simulink model "New_BMS_2"  (R2023b)
settings: Solver=FixedStepAuto  StartTime=0.0  StopTime=1000  FixedStep=0.1  RelTol=1e-3
InitFcn:
  | mbd_s32k_consistency_checks(bdroot(gcs));
undefined symbols (not defined in the file or in its folder): DiscIntNeverNeededParam, LQFP
libraries: mbd_s32k1xx_ec_toolbox x12, simulink x1
settings Model: Creator=snith  LastModifiedBy=HP
settings DataIOCC: ExternalInput=off  InitialState=off  SaveOutput=off  SignalLogging=off  SaveTime=off
settings OptimizationCC: DefaultParameterBehavior=Inlined  EnhancedBackFolding=on  PassReuseOutputArgsAs=Individual arguments  ZeroExternalMemoryAtStartup=off  ZeroInternalMemoryAtStartup=off  OptimizeBlockOrder=speed  DifferentSizesBufferReuse=on  OptimizationCustomize=off  EfficientTunableParamExpr=on
settings DebuggingCC: InheritedTsInSrcMsg=none  SingleTaskRateTransMsg=error  ParameterTunabilityLossMsg=error  UnconnectedInputMsg=error  UnconnectedOutputMsg=error  UnconnectedLineMsg=error  UnknownTsInhSupMsg=error
settings HardwareCC: ProdBitPerPointer=32  ProdBitPerSizeT=32  ProdBitPerPtrDiffT=32  ProdLargestAtomicInteger=Long  ProdLargestAtomicFloat=Double  ProdWordSize=32  ProdHWDeviceType=ARM Compatible->ARM Cortex
settings SFSimCC: MATLABDynamicMemAlloc=off
settings RTWCC: Description=Model Based Design Toolbox S32K1xx Code Generation Target  SystemTargetFile=mbd_s32k.tlc  MakeCommand=mbd_s32k_make_rtw COPY_MDLREF_INCLUDES=0  TemplateMakefile=mbd_s32k.tmf
settings CodeAppCC: ForceParamTrailComments=on  IgnoreCustomStorageClasses=off  OperatorAnnotations=on  SimulinkDataObjDesc=on  SFDataObjDesc=on  InsertBlockDesc=on
settings STFCustomTargetCC: MultiwordLength=256  CombineOutputUpdateFcns=on  ERTCustomFileBanners=on  SupportContinuousTime=off  SupportNonInlinedSFcns=off  RemoveResetFunc=on  MATLABClassNameForMDSCustomization=Simulink.SoftwareTarget.ERTCustomization  SystemTargetFile=mbd_s32k.tlc
settings ERTTargetCC: TargetLangStandard=C99 (ISO)  ParMdlRefBuildCompliant=off  CompOptLevelCompliant=off  ConcurrentExecutionCompliant=off  ModelStepFunctionPrototypeControlCompliant=off  CPPClassGenCompliant=off  UseToolchainInfoCompliant=off  InlinedParameterPlacement=NonHierarchical  ERTSrcFileBannerTemplate=mbd_ert_code_template.cgt  ERTHdrFileBannerTemplate=mbd_ert_code_template.cgt  ERTDataSrcFileTemplate=mbd_ert_code_template.cgt  ERTDataHdrFileTemplate=mbd_ert_code_template.cgt  ERTCustomFileTemplate=example_file_process.tlc
settings ConfigComp: CovBoundaryAbsTol=1.0e-5

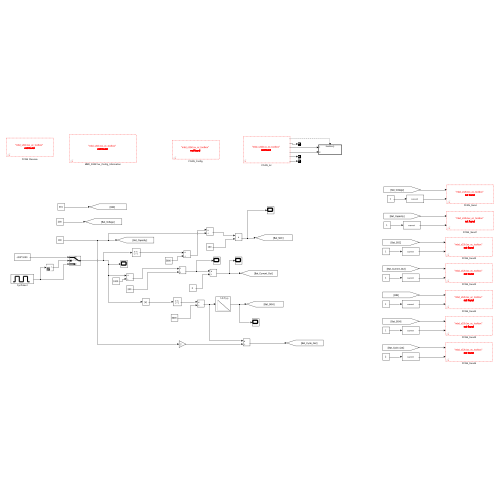
[thumbnail: Simulink's stored preview of the top-level diagram]
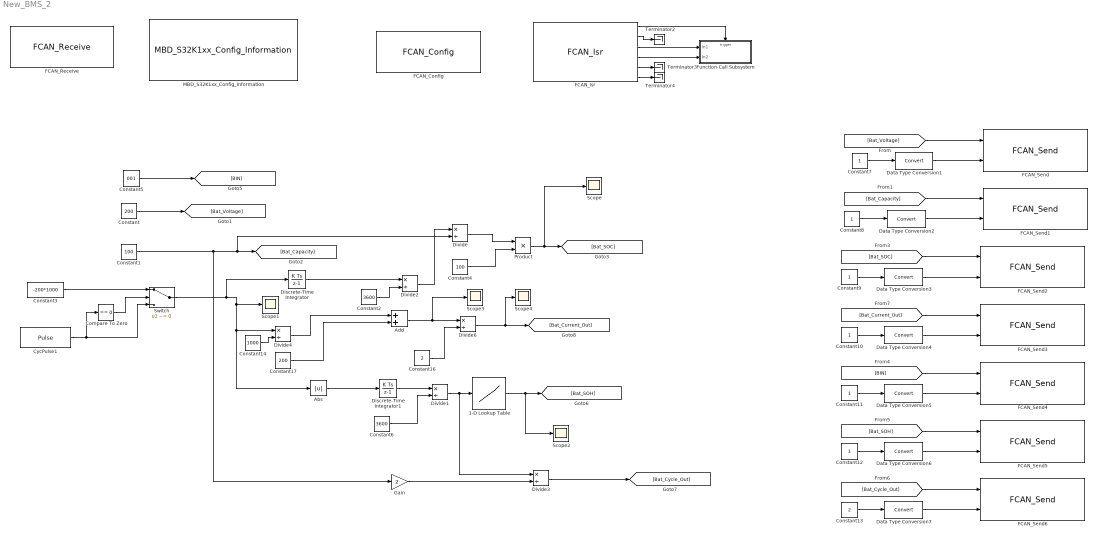
== system New_BMS_2 ==
  1-D Lookup Table : Lookup_n-D  NumberOfTableDimensions=1  BreakpointsForDimension1=[0 10000 20000 40000 60000 80000 100000 120000 140000 160000 180000]  Table=[100 99 98 96 94 92 90 88 86 84 82]  TableDataTypeStr=Inherit: Inherit from 'Table data'  ExtrapMethod=Clip  InternalRulePriority=Speed  OutDataTypeStr=uint8  RndMeth=Simplest
  Abs : Abs  SaturateOnIntegerOverflow=off
  Add : Sum  OutDataTypeStr=Inherit: Inherit via back propagation
  Compare To Zero : simulink/Logic and Bit Operations/Compare To Zero  relop===  OutDataTypeStr=boolean
  Constant : Constant  Value=200  OutDataTypeStr=uint8
  Constant1 : Constant  Value=100  OutDataTypeStr=uint8
  Constant{7..12} (6 alike) : Constant
  Constant13 : Constant  Value=2
  Constant14 : Constant  Value=1000
  Constant16 : Constant  Value=2
  Constant17 : Constant  Value=200
  Constant2 : Constant  Value=3600
  Constant3 : Constant  Value=-200*1000
  Constant4 : Constant  Value=100
  Constant5 : Constant  Value=001  OutDataTypeStr=uint8
  Constant6 : Constant  Value=3600
  CycPulse1 : DiscretePulseGenerator  PulseType=Time based  Amplitude=200*1000  Period=3600/1000  PulseWidth=50
  Data Type Conversion{1..7} (7 alike) : DataTypeConversion  SaturateOnIntegerOverflow=off  RndMeth=Floor
  Discrete-Time Integrator : DiscreteIntegrator  SampleTime=-1  ICPrevOutput=DiscIntNeverNeededParam  ICPrevScaledInput=DiscIntNeverNeededParam
  Discrete-Time Integrator1 : DiscreteIntegrator  SampleTime=-1  ICPrevOutput=DiscIntNeverNeededParam  ICPrevScaledInput=DiscIntNeverNeededParam
  Divide : Product  Inputs=*/
  Divide1 : Product  Inputs=*/
  Divide2 : Product  Inputs=*/
  Divide3 : Product  Inputs=*/  OutDataTypeStr=uint8
  Divide4 : Product  Inputs=*/  OutDataTypeStr=double
  Divide6 : Product  Inputs=*/  OutDataTypeStr=uint8
  FCAN_Config : mbd_s32k1xx_ec_toolbox/Communication Blocks/CAN Blocks/FCAN_Config  Priority=1  can_instance=0  can_mode=Normal mode  can_max_num_mb=20  can_rx=PTE4: [CAN0_RX | CAN Rx channel]  can_tx=PTE5: [CAN0_TX | CAN Tx Channel]  show_adv_opts=on  can_clk_src=Peripheral clock  can_clk_freq=80 MHz  bitrate_to_time_seg=on  bitrate=500  sample_point=80  real_bitrate=500  real_sample_point=80  prop_delay=250  bus_length=1  tq=200.0  time_quanta=10  can_presdiv=16  can_propseg=3  can_pseg1=4  can_pseg2=2  can_rjw=2  cbt_bitrate=2000  cbt_sample_point=80  cbt_real_bitrate=2000  cbt_real_sample_point=80  cbt_tq=25.0  cbt_time_quanta=40  can_cbt_presdiv=2  can_cbt_propseg=29  can_cbt_pseg1=5  can_cbt_pseg2=5  can_cbt_rjw=5  can_fd_enable=off  can_payload=8  tdc_enable=off  tdc_offset=20  can_rxfifo_enable=off  can_num_id_filters=8  can_fifo_id_format=A  can_fifo_id_filter={{false,false,'0x0'},{false,false,'0x0'},{false,false,'0x0'},{false,false,'0x0'},{false,false,'0x0'},{false,false,'0x0'},{false,false,'0x0'},{false,false,'0x0'}}  can_pn_enable=off  can_wakeup_match=off  can_wakeup_timeout=off  can_timeout_en=off  can_match_timeout=1  can_multiple_matches_en=off  can_num_matches=1  can_idfilter_extendedid=off  can_idfilter_remoteframe=off  can_idfilter_type=Match exact  can_idfilter_id1=0  can_idfilter_id2=0  can_payloadfilter_enable=off  can_payloadfilter_dlclow=0  can_payloadfilter_dlchigh=0  can_payloadfilter_type=Match exact  can_payloadfilter_payload1_b0=0  can_payloadfilter_payload1_b1=0  can_payloadfilter_payload1_b2=0  can_payloadfilter_payload1_b3=0  can_payloadfilter_payload1_b4=0  can_payloadfilter_payload1_b5=0  can_payloadfilter_payload1_b6=0  can_payloadfilter_payload1_b7=0  can_payloadfilter_payload2_b0=0  can_payloadfilter_payload2_b1=0  can_payloadfilter_payload2_b2=0  can_payloadfilter_payload2_b3=0  can_payloadfilter_payload2_b4=0  can_payloadfilter_payload2_b5=0  can_payloadfilter_payload2_b6=0  can_payloadfilter_payload2_b7=0
  FCAN_Isr : mbd_s32k1xx_ec_toolbox/Communication Blocks/CAN Blocks/FCAN_Isr  can_instance=0  can_event=Rx Complete
  FCAN_Receive : mbd_s32k1xx_ec_toolbox/Communication Blocks/CAN Blocks/FCAN_Receive  can_instance=0  can_mode=Non-blocking  can_timeout_ms=0  can_mb_idx=19  can_mb_init=Once  show_id_input=off  can_extended_id=off  can_is_remote=off  can_id=123  can_msg_mask=FFFFFFFF  show_adv_opts=off  can_use_rxfifo=off  can_fd_enable=off
  FCAN_Send : mbd_s32k1xx_ec_toolbox/Communication Blocks/CAN Blocks/FCAN_Send  can_instance=0  can_mode=Non-blocking  can_timeout_ms=0  can_mb_idx=10  can_mb_init=On each call  show_id_input=off  can_extended_id=off  can_is_remote=off  can_id=100  show_adv_opts=off  can_fd_enable=off  can_enable_brs=off  can_fd_padding=0
  FCAN_Send1 : mbd_s32k1xx_ec_toolbox/Communication Blocks/CAN Blocks/FCAN_Send  can_instance=0  can_mode=Non-blocking  can_timeout_ms=0  can_mb_idx=11  can_mb_init=On each call  show_id_input=off  can_extended_id=off  can_is_remote=off  can_id=101  show_adv_opts=off  can_fd_enable=off  can_enable_brs=off  can_fd_padding=0
  FCAN_Send2 : mbd_s32k1xx_ec_toolbox/Communication Blocks/CAN Blocks/FCAN_Send  can_instance=0  can_mode=Non-blocking  can_timeout_ms=0  can_mb_idx=12  can_mb_init=On each call  show_id_input=off  can_extended_id=off  can_is_remote=off  can_id=102  show_adv_opts=off  can_fd_enable=off  can_enable_brs=off  can_fd_padding=0
  FCAN_Send3 : mbd_s32k1xx_ec_toolbox/Communication Blocks/CAN Blocks/FCAN_Send  can_instance=0  can_mode=Non-blocking  can_timeout_ms=0  can_mb_idx=13  can_mb_init=On each call  show_id_input=off  can_extended_id=off  can_is_remote=off  can_id=103  show_adv_opts=off  can_fd_enable=off  can_enable_brs=off  can_fd_padding=0
  FCAN_Send4 : mbd_s32k1xx_ec_toolbox/Communication Blocks/CAN Blocks/FCAN_Send  can_instance=0  can_mode=Non-blocking  can_timeout_ms=0  can_mb_idx=14  can_mb_init=On each call  show_id_input=off  can_extended_id=off  can_is_remote=off  can_id=104  show_adv_opts=off  can_fd_enable=off  can_enable_brs=off  can_fd_padding=0
  FCAN_Send5 : mbd_s32k1xx_ec_toolbox/Communication Blocks/CAN Blocks/FCAN_Send  can_instance=0  can_mode=Non-blocking  can_timeout_ms=0  can_mb_idx=15  can_mb_init=On each call  show_id_input=off  can_extended_id=off  can_is_remote=off  can_id=105  show_adv_opts=off  can_fd_enable=off  can_enable_brs=off  can_fd_padding=0
  FCAN_Send6 : mbd_s32k1xx_ec_toolbox/Communication Blocks/CAN Blocks/FCAN_Send  can_instance=0  can_mode=Non-blocking  can_timeout_ms=0  can_mb_idx=16  can_mb_init=On each call  show_id_input=off  can_extended_id=off  can_is_remote=off  can_id=106  show_adv_opts=off  can_fd_enable=off  can_enable_brs=off  can_fd_padding=0
  Function-Call Subsystem : Subsystem  TreatAsAtomicUnit=on
  Gain : Gain  Gain=2
  MBD_S32K1xx_Config_Information : mbd_s32k1xx_ec_toolbox/MBD_S32K1xx_Config_Information  mbdt_ver=0  disp_str=|  config_params=[]  mcu_target_name=S32K144  mcu_target_package=100-LQFP  mcu_target_sram_size=48KB  mcu_system_clock_freq=80  mcu_xtal_freq=External 8  mcu_steptick_timer=LPIT Channel 0  mcu_steptick_prio=15  ds_import_enable=on  target_compiler=GCC  target_memory=FLASH  gcc_target_compile_opts=-mthumb -mfloat-abi=hard -mfpu=fpv4-sp-d16 -O1 -g -gstrict-dwarf  gcc_target_assemble_opts=-mthumb -mfloat-abi=hard -mfpu=fpv4-sp-d16 -g  gcc_target_link_opts=-mthumb -mfloat-abi=hard -mfpu=fpv4-sp-d16  gcc_target_default_lcf=on  gcc_target_user_lcf=S32K144_48_flash.ld  ghs_target_compile_opts=-cpu=cortexm4f -thumb -fpu=vfpv4_d16 -fsingle -Ogeneral -Wundef -Wimplicit-int -Wshadow -Wtrigraphs --no_commons --gnu_asm -gnu99 -gdwarf-2 -G  ghs_target_assemble_opts=-cpu=cortexm4f -fpu=vfpv4_d16  ghs_target_link_opts=-cpu=cortexm4f -thumb -fpu=vfpv4_d16  ghs_target_default_lcf=on  ghs_target_user_lcf=S32K144_48_flash.ld  iar_target_compile_opts=--cpu=Cortex-M4F --thumb --fpu=VFPv4_sp -Ol -e --debug --dlib_config normal  iar_target_assemble_opts=--cpu Cortex-M4F --thumb --fpu VFPv4_sp  iar_target_link_opts=--no_exceptions --vfe --inline  iar_target_default_lcf=on  iar_target_user_lcf=S32K144_48_flash.icf  pil_download_enable=on  rbl_download_enable=on  rbl_start_delay=5000  rbl_download_interface=JTAG  rbl_restart_request=off  rbl_com_port=Custom  rbl_com_port_custom=COM1  pil_download_rate=57600  pil_download_rate_custom=115200  pil_opensda_drive=Custom  pil_opensda_drive_custom=D  jtag_interface=SEGGER JLink  jlink_default_path=off  jlink_user_path=C:\NXP\S32DS.3.5\Drivers\Segger  pil_uart_instance=1  pil_uart_rx=PTC6: [LPUART1_RX | Receive]  pil_uart_tx=PTC7: [LPUART1_TX | Transmit]  FTM_PWM_PcrCheckEnDis=on  FTM_Input_Edge_Inputs_PcrCheckEnDis=on  FTM_Dual_Edge_Inputs_PcrCheckEnDis=on  FTM_Quadrature_Inputs_PcrCheckEnDis=on  FTM_Hall_Sensor_Inputs_PcrCheckEnDis=on  LPTMR_PcrCheckEnDis=on  PIT_PcrCheckEnDis=on  RTC_PcrCheckEnDis=on  FlexCAN_PcrCheckEnDis=on  LIN_PcrCheckEnDis=on  FlexIO_PcrCheckEnDis=on  LPI2C_PcrCheckEnDis=on  LPSPI_PcrCheckEnDis=on  LPUART_PcrCheckEnDis=on  CMP_PcrCheckEnDis=on  GPIO_OutputPcrCheckEnDis=on  GPIO_InputPcrCheckEnDis=on  SBC_PcrCheckEnDis=on  BMS_PcrCheckEnDis=on  AMMCLIB_PcrCheckEnDis=on  FM_PcrCheckEnDis=on  Profile_PcrCheckEnDis=on  ConfigParams_PcrCheckEnDis=on  ModelRef_PcrCheckEnDis=on  PDB0_PcrCheckEnDis=on  CSEc_PcrCheckEnDis=on  eDMA_PcrCheckEnDis=on  FLASH_PcrCheckEnDis=on  ADC_PcrCheckEnDis=on  WDOG_PcrCheckEnDis=on
      | Target : S32K144-64KB_SRAM
      | Package : 100-pin
      | System clock : 80 MHz
      | XTAL clock : External 8 MHz
      | Compiler : IAR
      | Target Type : FLASH
      | Download Code after build : off
      | Step Tick Interrupt Priority : 15
  Product : Product  OutDataTypeStr=uint8
  Scope{,1..4} (5 alike) : Scope
  Switch : Switch  Criteria=u2 ~= 0  OutDataTypeStr=Inherit: Inherit via back propagation  SaturateOnIntegerOverflow=off  InputSameDT=off
  Terminator2 : Terminator
  Terminator3 : Terminator
  Terminator4 : Terminator
  wires:
  Switch/1 -> Discrete-Time Integrator/1, Scope1/1, Divide4/1, Abs/1
  Divide/1 -> Product/1
  Discrete-Time Integrator1/1 -> Divide1/1
  CycPulse1/1 -> Compare To Zero/1, Switch/3
  1-D Lookup Table/1 -> [Bat_SOH], Scope2/1
  Constant1/1 -> [Bat_Capacity], Divide/2, Gain/1
  Constant5/1 -> [BIN]
  Constant4/1 -> Product/2
  Discrete-Time Integrator/1 -> Divide2/1
  Constant6/1 -> Divide1/2
  Constant2/1 -> Divide2/2
  Constant3/1 -> Switch/1
  Compare To Zero/1 -> Switch/2
  Abs/1 -> Discrete-Time Integrator1/1
  Product/1 -> Scope/1, [Bat_SOC]
  Divide1/1 -> Divide3/1, 1-D Lookup Table/1
  Divide2/1 -> Divide/1
  Constant7/1 -> Data Type Conversion1/1
  Data Type Conversion1/1 -> FCAN_Send/2
  Gain/1 -> Divide3/2
  FCAN_Isr/3 -> Function-Call Subsystem/1(In1)
  FCAN_Isr/1 -> Function-Call Subsystem/Trigger
  FCAN_Isr/4 -> Function-Call Subsystem/2(In2)
  FCAN_Isr/2 -> Terminator2/1
  FCAN_Isr/5 -> Terminator3/1
  FCAN_Isr/6 -> Terminator4/1
  Constant/1 -> [Bat_Voltage]
  [Bat_Voltage] -> FCAN_Send/1
  [Bat_Capacity] -> FCAN_Send1/1
  Data Type Conversion2/1 -> FCAN_Send1/2
  Constant8/1 -> Data Type Conversion2/1
  Data Type Conversion3/1 -> FCAN_Send2/2
  [Bat_SOC] -> FCAN_Send2/1
  Constant9/1 -> Data Type Conversion3/1
  [Bat_Current_Out] -> FCAN_Send3/1
  Data Type Conversion4/1 -> FCAN_Send3/2
  Constant10/1 -> Data Type Conversion4/1
  Constant11/1 -> Data Type Conversion5/1
  [BIN] -> FCAN_Send4/1
  Data Type Conversion5/1 -> FCAN_Send4/2
  [Bat_SOH] -> FCAN_Send5/1
  Constant12/1 -> Data Type Conversion6/1
  Data Type Conversion6/1 -> FCAN_Send5/2
  Constant13/1 -> Data Type Conversion7/1
  Data Type Conversion7/1 -> FCAN_Send6/2
  [Bat_Cycle_Out] -> FCAN_Send6/1
  Constant14/1 -> Divide4/2
  Divide4/1 -> Add/1
  Divide3/1 -> [Bat_Cycle_Out]
  Constant17/1 -> Add/2
  Constant16/1 -> Divide6/2
  Add/1 -> Scope3/1, Divide6/1
  Divide6/1 -> Scope4/1, [Bat_Current_Out]

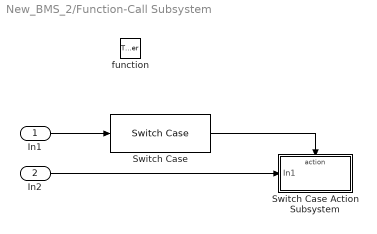
== system New_BMS_2/Function-Call Subsystem ==
  In1 : Inport
  In2 : Inport  Port=2
  function : TriggerPort  TriggerType=function-call  VariantControl=(inherit)
  Switch Case : SwitchCase  CaseConditions={hex2dec('123')}  ShowDefaultCase=off
  Switch Case Action Subsystem : Subsystem  TreatAsAtomicUnit=on
  wires:
  In1/1 -> Switch Case/1
  Switch Case/1 -> Switch Case Action Subsystem/Action
  In2/1 -> Switch Case Action Subsystem/1(In1)

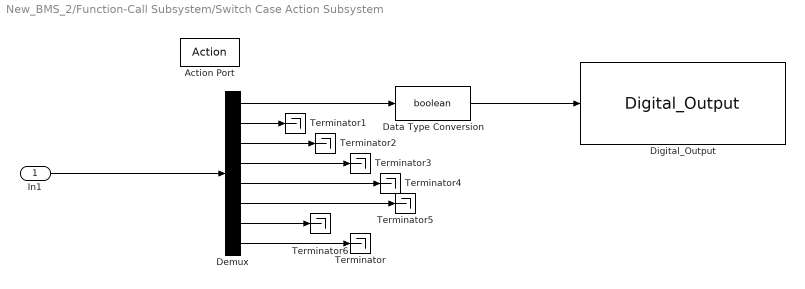
== system New_BMS_2/Function-Call Subsystem/Switch Case Action Subsystem ==
  In1 : Inport
  Action Port : ActionPort  ActionPortLabel=case [ 291 ]:
  Data Type Conversion : DataTypeConversion  OutDataTypeStr=boolean  SaturateOnIntegerOverflow=off  RndMeth=Floor
  Demux : Demux  Outputs=8
  Digital_Output : mbd_s32k1xx_ec_toolbox/GPIO Blocks/Digital_Output  gpio_pin=PTD15: [PTD15 | Port D I/O]  init_val=Low  drive_strength=Low
  Terminator{,1..6} (7 alike) : Terminator
  wires:
  In1/1 -> Demux/1
  Demux/1 -> Data Type Conversion/1
  Demux/8 -> Terminator/1
  Data Type Conversion/1 -> Digital_Output/1
  Demux/7 -> Terminator6/1
  Demux/6 -> Terminator5/1
  Demux/5 -> Terminator4/1
  Demux/4 -> Terminator3/1
  Demux/3 -> Terminator2/1
  Demux/2 -> Terminator1/1
